simulink library "AP_Connector"  (R2024b)
settings: Solver=VariableStepAuto  StartTime=0.0  StopTime=10.0  RelTol=1e-3
undefined symbols (not defined in the file or in its folder): dt
settings Model: Creator=Peter  LastModifiedBy=pcl
settings SolverCC: AlgebraicLoopSolver=TrustRegion
settings DebuggingCC: UnconnectedInputMsg=warning  UnconnectedOutputMsg=warning  UnconnectedLineMsg=warning
settings ModelReferenceCC: EnableRefExpFcnMdlSchedulingChecks=on
settings RTWCC: GPUComputeCapability=3.5

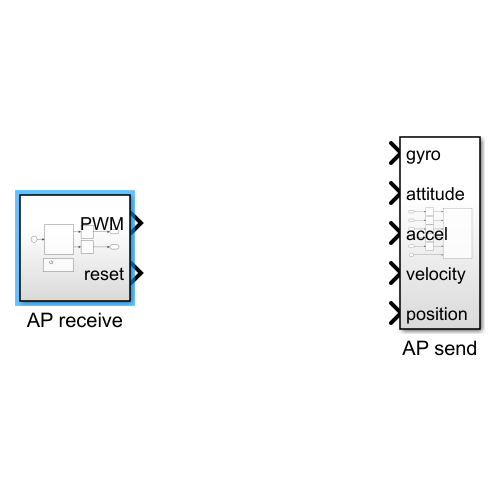
[thumbnail: Simulink's stored preview of the top-level diagram]
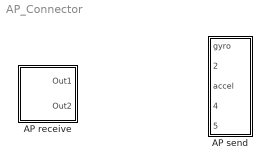
== system AP_Connector ==
  AP receive : Subsystem
  AP send : Subsystem

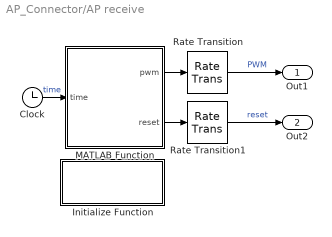
== system AP_Connector/AP receive ==
  Clock : Clock
  Initialize Function : Subsystem  TreatAsAtomicUnit=on
  MATLAB Function : MATLAB Function  TreatAsAtomicUnit=on  SystemSampleTime=dt
  Rate Transition : RateTransition
  Rate Transition1 : RateTransition
  Out1 : Outport
  Out2 : Outport  Port=2
  wires:
  Rate Transition/1 -> Out1/1  "PWM"
  MATLAB Function/1(pwm) -> Rate Transition/1
  Clock/1 -> MATLAB Function/1(time)  "time"
  MATLAB Function/2(reset) -> Rate Transition1/1
  Rate Transition1/1 -> Out2/1  "reset"

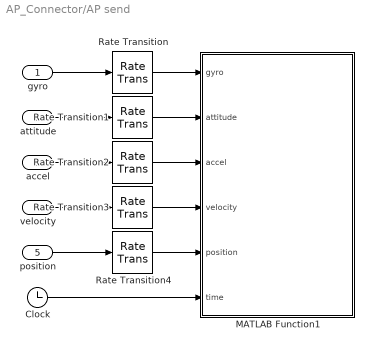
== system AP_Connector/AP send ==
  gyro : Inport
  attitude : Inport  Port=2
  accel : Inport  Port=3
  velocity : Inport  Port=4
  position : Inport  Port=5
  Clock : Clock
  MATLAB Function1 : MATLAB Function  TreatAsAtomicUnit=on  SystemSampleTime=dt
  Rate Transition{,1..4} (5 alike) : RateTransition
  wires:
  attitude/1 -> Rate Transition1/1
  gyro/1 -> Rate Transition/1
  Rate Transition/1 -> MATLAB Function1/1(gyro)
  Clock/1 -> MATLAB Function1/6(time)
  Rate Transition3/1 -> MATLAB Function1/4(velocity)
  Rate Transition2/1 -> MATLAB Function1/3(accel)
  Rate Transition1/1 -> MATLAB Function1/2(attitude)
  accel/1 -> Rate Transition2/1
  Rate Transition4/1 -> MATLAB Function1/5(position)
  velocity/1 -> Rate Transition3/1
  position/1 -> Rate Transition4/1

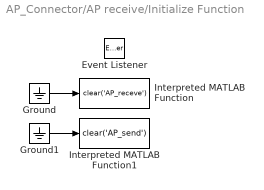
== system AP_Connector/AP receive/Initialize Function ==
  Event Listener : EventListener  DisableCoverage=on  EventName=reset
  Ground : Ground
  Ground1 : Ground
  Interpreted MATLAB Function : MATLABFcn  MATLABFcn=clear('AP_receve')  OutputDimensions=0
  Interpreted MATLAB Function1 : MATLABFcn  MATLABFcn=clear('AP_send')  OutputDimensions=0
  wires:
  Ground1/1 -> Interpreted MATLAB Function1/1
  Ground/1 -> Interpreted MATLAB Function/1

== matlab function AP_Connector/AP receive/MATLAB Function ==
  data: pwm output; time input; reset output
function [pwm, reset]  = fcn(time)
pwm = zeros(16,1); %#ok<PREALL>
reset = false; %#ok<NASGU>
coder.extrinsic('AP_receive')
[pwm, reset] = AP_receive(time);
end

== matlab function AP_Connector/AP send/MATLAB Function1 ==
  data: gyro input; attitude input; accel input; velocity input; position input; time input
function fcn(gyro, attitude, accel, velocity, position, time)
coder.extrinsic('AP_send')
AP_send(gyro, attitude, accel, velocity, position, time)
end
